simulink subsystem "Shooter_Controls_sub"  (R2023b)
settings: Solver=VariableStepAuto  StartTime=0.0  StopTime=10.0  RelTol=1e-3
undefined symbols (not defined in the file): Feeder_Max_Pulsetime, Field_BlueAllianceZoneX, Field_RedAllianceZoneX, Rebuilt_Feeder_Motor_Gain_FF, Rebuilt_Feeder_Time_FWD, Rebuilt_Feeder_Time_REV, Rebuilt_Hood_Servo_Pos_Min, Rebuilt_Match_Time_Auto_Timer, Rebuilt_Match_Time_End_Game_Timer, Rebuilt_Match_Time_Shift_1, Rebuilt_Match_Time_Shift_2, Rebuilt_Match_Time_Shift_3, Rebuilt_Match_Time_Shift_4, Rebuilt_Match_Time_Shift_Timer, Rebuilt_Match_Time_Shoot_Early, Rebuilt_Match_Time_Transition, Rebuilt_Negative_Feeder_Speed, Rebuilt_Shoot_Hood_Pos_Max_Error, Rebuilt_Shoot_Motor_Max_Error, Rebuilt_Shoot_Robot_Velocity_Max, Rebuilt_Shooter_Error_Integral_Enable, Rebuilt_Shooter_Motor_Gain_FF, Rebuilt_Shooter_Motor_Gain_I, Rebuilt_Shooter_Motor_Gain_I_Low, Rebuilt_Shooter_Motor_Gain_P, Rebuilt_Target_Feeder_Speed, Rebuilt_Target_Transfer_Speed, Rebuilt_Transfer_Error_Integral_Enable, Rebuilt_Transfer_Minimum_Factor, t_sample
libraries: simulink x20, Controls_Components_lib x2
(part 2 of 2)

== system Shooter_Controls_sub/Ready_to_Shoot/Check if allowed to score in alliance zone/Blue ==
  isBlueHubActive : Inport
  Robot_Position_X : Inport  Port=2
  Action Port : ActionPort
  AND : Logic  AllPortsSameDT=off  OutDataTypeStr=boolean
  BlueAllianceZoneX : Constant  Value=Field_BlueAllianceZoneX
  Less Than : RelationalOperator  Operator=<  OutDataTypeStr=boolean  RndMeth=Simplest  InputSameDT=off
  CanShootBlue : Outport
  wires:
  AND/1 -> CanShootBlue/1  "CanShootBlue"
  isBlueHubActive/1 -> AND/1
  Less Than/1 -> AND/2
  BlueAllianceZoneX/1 -> Less Than/2
  Robot_Position_X/1 -> Less Than/1

== system Shooter_Controls_sub/Ready_to_Shoot/Check if allowed to score in alliance zone/Red ==
  isRedHubActive : Inport
  Robot_Position_X : Inport  Port=2
  Action Port : ActionPort
  AND : Logic  AllPortsSameDT=off  OutDataTypeStr=boolean
  GreaterThan : RelationalOperator  Operator=>  OutDataTypeStr=boolean  RndMeth=Simplest  InputSameDT=off
  RedAllianceZoneX : Constant  Value=Field_RedAllianceZoneX
  CanShootRed : Outport
  wires:
  isRedHubActive/1 -> AND/1
  GreaterThan/1 -> AND/2
  AND/1 -> CanShootRed/1  "CanShootRed"
  RedAllianceZoneX/1 -> GreaterThan/2
  Robot_Position_X/1 -> GreaterThan/1

== system Shooter_Controls_sub/Ready_to_Shoot/Check if outside alliance zone/Blue ==
  Robot_Position_X1 : Inport
  Action Port : ActionPort
  BlueAllianceZoneX : Constant  Value=Field_BlueAllianceZoneX
  GreaterThan : RelationalOperator  Operator=>  OutDataTypeStr=boolean  RndMeth=Simplest  InputSameDT=off
  Can_Pass_Blue : Outport
  wires:
  GreaterThan/1 -> Can_Pass_Blue/1  "Can_Pass_Blue"
  Robot_Position_X1/1 -> GreaterThan/1
  BlueAllianceZoneX/1 -> GreaterThan/2

== system Shooter_Controls_sub/Ready_to_Shoot/Check if outside alliance zone/Red ==
  Robot_Position_X : Inport
  Action Port : ActionPort
  GreaterThan : RelationalOperator  Operator=<  OutDataTypeStr=boolean  RndMeth=Simplest  InputSameDT=off
  RedAllianceZoneX : Constant  Value=Field_RedAllianceZoneX
  Can_Pass_Red : Outport
  wires:
  GreaterThan/1 -> Can_Pass_Red/1  "Can_Pass_Red"
  RedAllianceZoneX/1 -> GreaterThan/2
  Robot_Position_X/1 -> GreaterThan/1

== stateflow chart Shooter_Controls_sub/Shooter_Transfer_Feeder Chart ==
  state Not_Shooting
    entry: Shooter_Active = false;
    Desired_Transfer_Speed = 0;
    Desired_Feeder_Speed = 0;
    Transfer_Initializing = 0;
  state Shooting
    entry: Shooter_Active = true;
    state Spinning_Up
      entry: Desired_Transfer_Speed = 0;
      Desired_Feeder_Speed = 0;
      Transfer_Initializing = 1;
    state Transfer
      entry: Desired_Feeder_Speed = Rebuilt_Negative_Feeder_Speed;
      Desired_Transfer_Speed = Rebuilt_Target_Transfer_Speed;
    state Feeder
      entry: Desired_Feeder_Speed = Rebuilt_Target_Feeder_Speed;
      Transfer_Initializing = 0;
      Feeder_Loops_Shooting = 0;
      during:
      Feeder_Loops_Shooting = Feeder_Loops_Shooting + 1;
    (default) -> Spinning_Up
    (junction 16) -> Spinning_Up : [(~Button_Shoot_Enable && ~Button_Unload_Manual) || ...
        | (Feeder_Loops_Shooting * t_sample > Feeder_Max_Pulsetime) || ...
        | (~Ready_to_Score && ~Ready_to_Pass && ~Ready_to_Unload_Manual)]
    (junction 14) -> (junction 16)
    Spinning_Up -> Transfer : [(Button_Shoot_Enable && (Ready_to_Score || Ready_to_Pass)) || ...
        | (Button_Unload_Manual && Ready_to_Unload_Manual)]
    Transfer -> (junction 14) [order 2]
    (junction 15) -> (junction 14)
    Transfer -> Feeder [order 1] : [Measured_Transfer_Speed > ...
        | Desired_Transfer_Speed * Rebuilt_Transfer_Minimum_Factor]
    Feeder -> (junction 15)
  (default) -> Not_Shooting
  Not_Shooting -> Shooting : [Button_Spinup_Enable || ...
      | Button_Shoot_Enable || ...
      | Button_Unload_Manual]
  Shooting -> Not_Shooting : [~Button_Spinup_Enable && ...
      | ~Button_Shoot_Enable && ...
      | ~Button_Unload_Manual]
  data: Rebuilt_Target_Transfer_Speed parameter; Measured_Transfer_Speed input; Rebuilt_Transfer_Minimum_Factor parameter; Ready_to_Score input; Button_Spinup_Enable input; Rebuilt_Target_Feeder_Speed parameter; Button_Shoot_Enable input; Button_Unload_Manual input; Shooter_Active output; Desired_Feeder_Speed output; Desired_Transfer_Speed output; Ready_to_Pass input; Rebuilt_Negative_Feeder_Speed parameter; Transfer_Initializing output; Feeder_Max_Pulsetime parameter; Feeder_Loops_Shooting local; t_sample parameter; Ready_to_Unload_Manual input

== stateflow chart Shooter_Controls_sub/Chart ==
  state if_reverse_or_zero
    entry: Desired_Feeder_Speed_Out = Desired_Feeder_Speed_In
    during: Desired_Feeder_Speed_Out = Desired_Feeder_Speed_In
  state if_forward
    state Forwards
      entry: Desired_Feeder_Speed_Out = Rebuilt_Target_Feeder_Speed;
    state Backwards
      entry: Desired_Feeder_Speed_Out = Rebuilt_Negative_Feeder_Speed;
    (default) -> Forwards
    Backwards -> Forwards : after(Rebuilt_Feeder_Time_REV, sec)
    Forwards -> Backwards : after(Rebuilt_Feeder_Time_FWD, sec)
  (default) -> if_reverse_or_zero
  if_reverse_or_zero -> if_forward : [(Desired_Feeder_Speed_In == Rebuilt_Target_Feeder_Speed) && Gamepad_Start]
  if_forward -> if_reverse_or_zero : [(Desired_Feeder_Speed_In == 0) || ~Gamepad_Start]
  data: Desired_Feeder_Speed_In input; Desired_Feeder_Speed_Out output; Rebuilt_Negative_Feeder_Speed parameter double; Rebuilt_Target_Feeder_Speed parameter double; Rebuilt_Feeder_Time_REV parameter; Rebuilt_Feeder_Time_FWD parameter; Gamepad_Start input boolean
